simulink model "rotpen_hardware_updown"  (R2025a)
settings: Solver=FixedStepAuto  StopTime=cycles*period  FixedStep=0.002  AbsTol=1e-3  EnableMultiTasking=on
values from neighbouring files (symbols this model uses):
  period = 7    [setup_updown.m]    (also in train_updown.m)
  phi0 = pi    (= 3.14159265359)    [setup_updown.m]    (also in train_updown.m)
  theta_limit = pi/2    (= 1.57079632679)    [setup_updown.m]    (also in train_updown.m)
  Ts = 0.01    [setup_updown.m]    (also in train_updown.m)
  volt_limit = 6    [setup_updown.m]    (also in train_updown.m)
undefined symbols (not defined in the file or in its folder): HIL, qc_get_step_size
libraries: quarc_library x3, simulink x2, rllib x1
settings Model: SimulationMode=accelerator  Creator=The MathWorks, Inc.  LastModifiedBy=liam
settings SolverCC: AutoScaleAbsTol=off  PositivePriorityOrder=on  AutoInsertRateTranBlk=on  MaxZcPerStep=1.0
settings DataIOCC: SaveOutput=off  SaveTime=off
settings DebuggingCC: UnconnectedInputMsg=warning  UnconnectedOutputMsg=warning  UnconnectedLineMsg=warning
settings ModelReferenceCC: EnableRefExpFcnMdlSchedulingChecks=on
settings RTWCC: SystemTargetFile=quarc_win64.tlc  Toolchain=QUARC win64 | nmake (64-bit Windows)  BuildConfiguration=Faster Runs  GPUComputeCapability=3.5  DLArmComputeVersion=19.05  Description=QUARC Win64 Target Using Toolchain
settings STFCustomTargetCC: SystemTargetFile=quarc_win64.tlc  MultiwordLength=2048.0  ConcurrentExecutionCompliant=on  UseToolchainInfoCompliant=on
settings GRTTargetCC: ExtMode=on  ExtModeMexFile=quarc_comm  ParMdlRefBuildCompliant=off  CompOptLevelCompliant=off  CombineOutputUpdateFcns=off  MatFileLogging=off  CPPClassGenCompliant=off  GRTInterface=on
settings ExplorerConfigSet: SimMechanicsOpenEditorOnUpdate=off  InternalSimMechanicsExplorerSettings="<ExplorerConfiguration><canonicalview>default</canonicalview><AnimationSetting><BasePlaybackSpeed>1.0</BasePlaybackSpeed><PlaybackSpeedFactor>1.0</PlaybackSpeedFactor></AnimationSetting><TilePanel><TileInfo><Tiles Columns=\"1\" Count=\"1\" Rows=\"1\"><Column Weight=\"1\"/><Row Weight=\"1\"/><Tile Height=\"1\" Width=\"1\" X=\"0\" Y=\"0\"/></Tiles></TileInfo><SceneInfo><SceneViewer><BGColor><R>0.60000002384185791</R><G>0.60000002384185791</G><B>0.60000002384185791</B></BGColor><Camera><DoPerspective>on</DoPerspective><Position><X>0.334156231583514596</X><Y>0.107146061295956732</Y><Z>0.154419804164132285</Z></Position><Center><X>0.145480827141795971</X><Y>0.0537418892551446009</Y><Z>0.077934111254939889</Z></Center><Up><X>-0.332530024195597795</X><Y>-0.157027945704575345</Y><Z>0.929927958110882913</Z></Up><ViewLimDist>1</ViewLimDist><YLim>0.466307658154998583</YLim><XLim>0.535390274177961367</XLim></Camera></SceneViewer></SceneInfo></TilePanel><MechEditorPanel><Cameras><Camera><Id>Camera1</Id><Value><Name>Camera1</Name><NativeCamera><PositionKeyframeSet/><CenterKeyframeSet/><UpVectorKeyframeSet/></NativeCamera></Value></Camera></Cameras><GfxPanelCameraMap><MapElement CameraMLId=\"Camera1\" GfxPanelIndex=\"0\"/></GfxPanelCameraMap><VideoCreator><PlaybackSpeedRatio>1.0</PlaybackSpeedRatio><FrameRate>30</FrameRate><VideoFormat>Motion JPEG AVI</VideoFormat><FrameSize>auto</FrameSize></VideoCreator></MechEditorPanel></ExplorerConfiguration>"

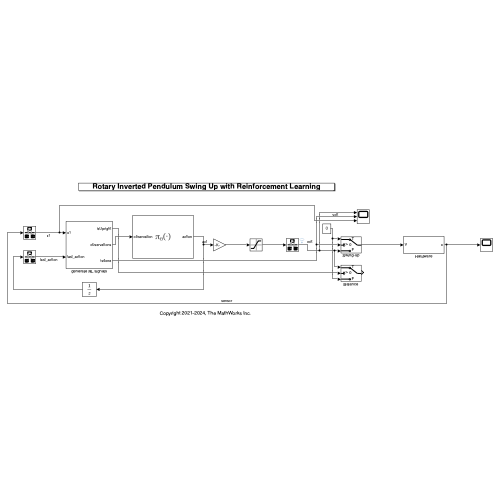
[thumbnail: Simulink's stored preview of the top-level diagram]
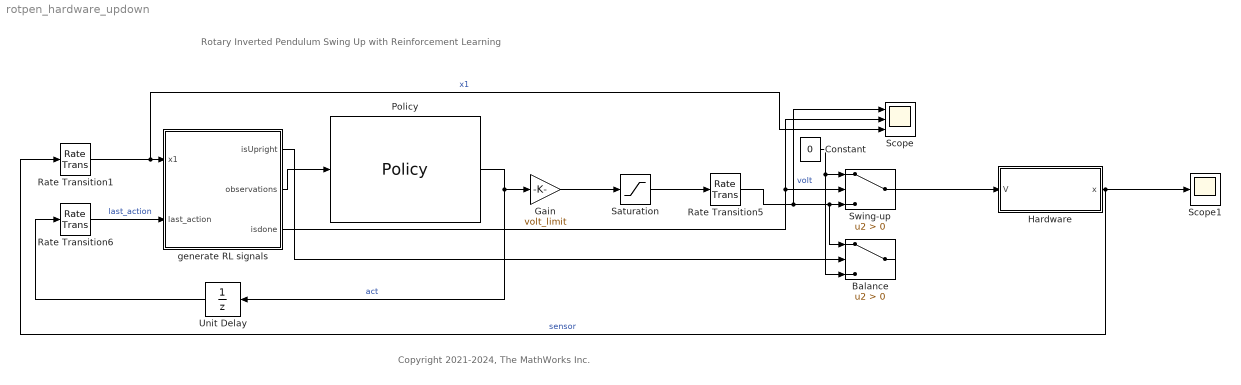
== system rotpen_hardware_updown ==
  note: Rotary Inverted Pendulum Swing Up with Reinforcement Learning
  note: Copyright 2021-2024, The MathWorks Inc.
  Balance : Switch  Criteria=u2 > Threshold  SaturateOnIntegerOverflow=off  InputSameDT=off
  Constant : Constant  Value=0
  Gain : Gain  Gain=volt_limit
  Hardware : Subsystem
  Policy : rllib/Policy  MATFile=updown_policy.mat  PolicyParamsAsInput=off  PolicyParamsBusName=policy_param_bus  SimUsingCodegen=off
  Rate Transition1 : RateTransition  OutPortSampleTime=Ts
  Rate Transition5 : RateTransition  OutPortSampleTime=Ts
  Rate Transition6 : RateTransition  OutPortSampleTime=Ts
  Saturation : Saturate  UpperLimit=8  LowerLimit=-8
  Scope : Scope  NumInputPorts=3
      settings: ActiveDisplayYMinimum=-16.085120303144286  ActiveDisplayYMaximum=13.822735216201398  DataLoggingVariableName=ScopeData2
  Scope1 : Scope
      settings: ActiveDisplayYMinimum=-19.051532422522097  ActiveDisplayYMaximum=18.818428112302271
  Swing-up : Switch  Criteria=u2 > Threshold  SaturateOnIntegerOverflow=off  InputSameDT=off
  Unit Delay : UnitDelay  SampleTime=-1
  generate RL signals : Subsystem
  wires:
  generate RL signals/3(isdone) -> Scope/2, Swing-up/2
  Policy/1 -> Gain/1, Unit Delay/1  "act"
  generate RL signals/2(observations) -> Policy/1
  Rate Transition1/1 -> Scope/3, generate RL signals/1(x1)  "x1"
  Unit Delay/1 -> Rate Transition6/1
  Hardware/1(x) -> Rate Transition1/1, Scope1/1  "sensor"
  Rate Transition6/1 -> generate RL signals/2(last_action)  "last_action"
  Saturation/1 -> Rate Transition5/1
  Rate Transition5/1 -> Balance/1, Swing-up/3, Scope/1  "volt"
  Constant/1 -> Swing-up/1, Balance/3
  generate RL signals/1(isUpright) -> Balance/2
  Gain/1 -> Saturation/1
  Swing-up/1 -> Hardware/1(V)

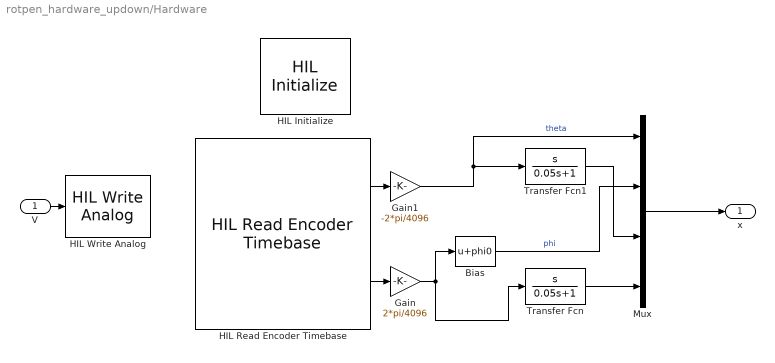
== system rotpen_hardware_updown/Hardware ==
  V : Inport
  Bias : Bias  Bias=phi0  SaturateOnIntegerOverflow=off
  Gain : Gain  Gain=2*pi/4096
  Gain1 : Gain  Gain=-2*pi/4096
  HIL Initialize : quarc_library/Data Acquisition/Generic/Configuration/HIL Initialize  object_name=HIL-1  board_type=q2_usb  board_number=0  board_options=d0=digital;d1=digital;led=auto;update_rate=normal;decimation=1  exclusive=off  active=on  hardware_clocks=[0]  clock_modes=[]  initial_clock_frequencies=[]  set_clock_params_at_start=off  set_clock_params_at_switch_in=off  set_clock_frequencies_at_start=off  set_clock_frequencies_at_switch_in=off  analog_input_channels=[0:1]  analog_input_configurations=[]  analog_input_maximums=10  analog_input_minimums=-10  set_analog_input_params_at_start=on  set_analog_input_params_at_switch_in=off  analog_output_channels=[0:1]  analog_output_maximums=10  analog_output_minimums=-10  initial_analog_outputs=[0]  final_analog_outputs=[0]  watchdog_analog_outputs=0  set_analog_output_params_at_start=on  set_analog_output_params_at_switch_in=off  set_analog_outputs_at_start=on  set_analog_outputs_at_switch_in=off  set_analog_outputs_at_terminate=on  set_analog_outputs_at_switch_out=off  set_analog_outputs_on_watchdog=off  digital_input_channels=[]  digital_output_channels=[]  digital_output_configuration=[]  initial_digital_outputs=[1]  final_digital_outputs=[1]  watchdog_digital_outputs=[1]  set_digital_output_params_at_start=off  set_digital_output_params_at_switch_in=off  set_digital_outputs_at_start=on  set_digital_outputs_at_switch_in=off  set_digital_outputs_at_terminate=on  set_digital_outputs_at_switch_out=off  set_digital_outputs_on_watchdog=off  encoder_channels=[0:1]  quadrature=[4]  encoder_filter_frequency=[]  initial_encoder_counts=[0]  set_encoder_params_at_start=on  set_encoder_params_at_switch_in=off  set_encoder_counts_at_start=on  set_encoder_counts_at_switch_in=off  pwm_channels=[]  pwm_modes=[0]  pwm_frequency=1/0.020  pwm_configuration=[]  pwm_alignment=[]  pwm_polarity=[]  pwm_leading_deadband=[]  pwm_trailing_deadband=[]  initial_pwm_outputs=[0]  final_pwm_outputs=[0]  watchdog_pwm_outputs=[0]  set_pwm_params_at_start=on  set_pwm_params_at_switch_in=off  set_pwm_outputs_at_start=on  set_pwm_outputs_at_switch_in=off  set_pwm_outputs_at_terminate=on  set_pwm_outputs_at_switch_out=off  set_pwm_outputs_on_watchdog=off  other_output_channels=[]  initial_other_outputs=[]  final_other_outputs=[]  watchdog_other_outputs=[]  set_other_outputs_at_start=off  set_other_outputs_at_switch_in=off  set_other_outputs_at_terminate=off  set_other_outputs_at_switch_out=off  set_other_outputs_on_watchdog=off
  HIL Read Encoder Timebase : quarc_library/Data Acquisition/Generic/Timebases/HIL Read Encoder Timebase  object_name=HIL-1  clock=0  channels=[0 1]  active=on  vector_output=off  data_type_mode=Inherit via back propagation  data_type=double  overflow_mode=Error on overflow  samples_in_buffer=max(ceil(1/qc_get_step_size), 1)
  HIL Write Analog : quarc_library/Data Acquisition/Generic/Immediate I//O/HIL Write Analog  object_name=HIL-1  channels=0  sample_time=-1  active=off  vector_input=off
  Mux : Mux
  Transfer Fcn : TransferFcn  Numerator=[1 0]  Denominator=[0.05 1]
  Transfer Fcn1 : TransferFcn  Numerator=[1 0]  Denominator=[0.05 1]
  x : Outport
  wires:
  V/1 -> HIL Write Analog/1
  HIL Read Encoder Timebase/1 -> Gain1/1
  HIL Read Encoder Timebase/2 -> Gain/1
  Gain1/1 -> Mux/1, Transfer Fcn1/1  "theta"
  Gain/1 -> Transfer Fcn/1, Bias/1
  Bias/1 -> Mux/2  "phi"
  Transfer Fcn1/1 -> Mux/3
  Transfer Fcn/1 -> Mux/4
  Mux/1 -> x/1

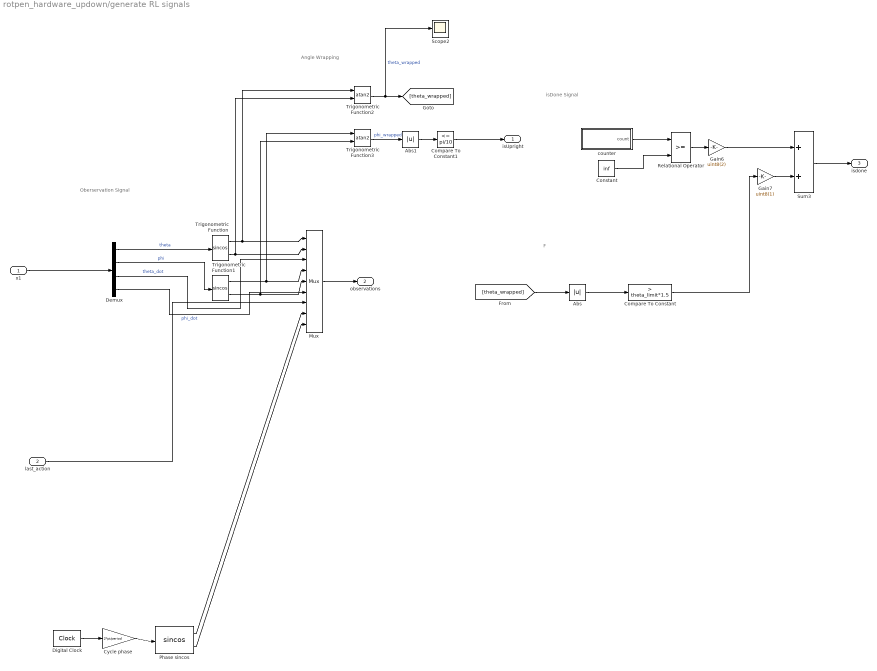
== system rotpen_hardware_updown/generate RL signals ==
  note: Oberservation Signal
  note: isDone Signal
  note: Angle Wrapping
  note: F
  x1 : Inport  SampleTime=Ts
  last_action : Inport  Port=2
  Abs : Abs  SaturateOnIntegerOverflow=off
  Abs1 : Abs  SaturateOnIntegerOverflow=off
  Compare To Constant : simulink/Logic and Bit Operations/Compare To Constant  relop=>  const=theta_limit*1.5  OutDataTypeStr=boolean
  Compare To Constant1 : simulink/Logic and Bit Operations/Compare To Constant  relop=<=  const=pi/10  OutDataTypeStr=boolean
  Constant : Constant  Value=inf
  Cycle phase : Gain  Gain=2*pi/period
  Demux : Demux
  Digital Clock : DigitalClock  SampleTime=Ts
  Gain6 : Gain  Gain=uint8(2)  OutDataTypeStr=uint8
  Gain7 : Gain  Gain=uint8(1)  OutDataTypeStr=uint8
  Mux : Mux  Inputs=9
  Phase sincos : Trigonometry  Operator=sincos
  Relational Operator : RelationalOperator  OutDataTypeStr=boolean  RndMeth=Simplest  InputSameDT=off
  Scope2 : Scope
      settings: ActiveDisplayYMinimum=-3.8840393549264434  ActiveDisplayYMaximum=3.8932432396537573  DataLoggingVariableName=ScopeData3
  Sum3 : Sum
  Trigonometric Function : Trigonometry  Operator=sincos
  Trigonometric Function1 : Trigonometry  Operator=sincos
  Trigonometric Function2 : Trigonometry  Operator=atan2
  Trigonometric Function3 : Trigonometry  Operator=atan2
  counter : Subsystem
  isUpright : Outport
  observations : Outport  Port=2
  isdone : Outport  Port=3
  wires:
  Trigonometric Function1/1 -> Trigonometric Function3/1, Mux/4
  Trigonometric Function2/1 -> Scope2/1, [theta_wrapped]  "theta_wrapped"
  Mux/1 -> observations/1
  Trigonometric Function1/2 -> Trigonometric Function3/2, Mux/5
  counter/1(count) -> Relational Operator/1
  Trigonometric Function/2 -> Trigonometric Function2/2, Mux/2
  x1/1 -> Demux/1
  Relational Operator/1 -> Gain6/1
  Constant/1 -> Relational Operator/2
  Sum3/1 -> isdone/1
  Trigonometric Function/1 -> Trigonometric Function2/1, Mux/1
  Abs/1 -> Compare To Constant/1
  [theta_wrapped] -> Abs/1
  last_action/1 -> Mux/7
  Trigonometric Function3/1 -> Abs1/1  "phi_wrapped"
  Gain6/1 -> Sum3/1
  Gain7/1 -> Sum3/2
  Demux/4 -> Mux/6  "phi_dot"
  Compare To Constant/1 -> Gain7/1
  Demux/1 -> Trigonometric Function/1  "theta"
  Demux/2 -> Trigonometric Function1/1  "phi"
  Demux/3 -> Mux/3  "theta_dot"
  Abs1/1 -> Compare To Constant1/1
  Compare To Constant1/1 -> isUpright/1
  Digital Clock/1 -> Cycle phase/1
  Cycle phase/1 -> Phase sincos/1
  Phase sincos/1 -> Mux/8
  Phase sincos/2 -> Mux/9

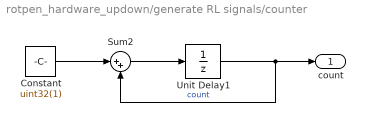
== system rotpen_hardware_updown/generate RL signals/counter ==
  Constant : Constant  Value=uint32(1)
  Sum2 : Sum  Inputs=|++
  Unit Delay1 : UnitDelay  SampleTime=Ts
  count : Outport  OutDataTypeStr=uint32
  wires:
  Sum2/1 -> Unit Delay1/1
  Unit Delay1/1 -> count/1, Sum2/2  "count"
  Constant/1 -> Sum2/1
